simulink model "Simulink_DC_MG_4DGs_4Lines"  (R2024a)
settings: Solver=VariableStepAuto  StartTime=0.0  StopTime=10  RelTol=1e-3
InitFcn:
  | % In your simulation loop or callback function
  | for l = 1:numOfLines
  |     % Generate resistance disturbance (10% variation)
  |     delta_R_l = 0.1 * randn() * Line{l}.R;
  | 
  |     % Update the line resistance with disturbance
  |     Line{l}.R_disturbed = Line{l}.R + delta_R_l;
  | 
  |     % Use this disturbed value in your simulation equations
  |     % L_l * dI_l/dt = -Line{l}.R_disturbed * I_l + (V_i - V_j)
  | end
values from neighbouring files (symbols this model uses):
  Is = value(Is)    [implementTheorem1.m]    (also in implementTheorem1_Obj.m; implementTheorem1_debug.m = []; implementTheorem1_minLoss.m)
  K = sdpvar(1, 3, 'full')    [ComputePassivityForDGs.m]
  l = lines(k, 2)    [generatePhysicalTopology.m]    (also in ploting.m = legend({'\bf With Disturbance'},     'Location','southeast',)
  numOfDGs = size(B_il,1)    [centralizedLocalControlDesign.m]    (also in generateCommunicationTopology.m = size(coords, 1); globalControlDesign.m = size(B_il, 1); verifyControlConditions.m)
undefined symbols (not defined in the file or in its folder): Current_Load_activation, current_variance, D_Activation, DC_Activation, DG, LC_Activation, Line, line_variance, PlugIn, PlugOut, SS_Activation, V_nom, V_ref, voltage_variance
libraries: spsSeriesRLCBranchLib x28, spsControlledCurrentSourceLib x12, spsCurrentMeasurementLib x8, simulink x4, spsIdealSwitchLib x4, spsStairGeneratorLib x4, spsControlledVoltageSourceLib x4, spsDCVoltageSourceLib x4, spsDiodeLib x4, spsIGBTLib x4, spsVoltageMeasurementLib x4, spspowerguiLib x1
(part 1 of 2)
settings Model: Creator=najaf  LastModifiedBy=najaf
settings RTWCC: GPUComputeCapability=3.5

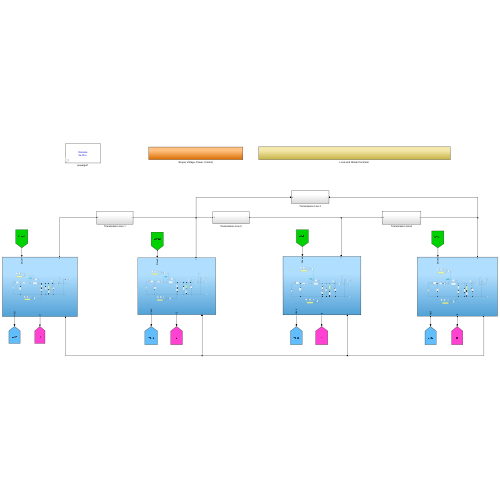
[thumbnail: Simulink's stored preview of the top-level diagram]
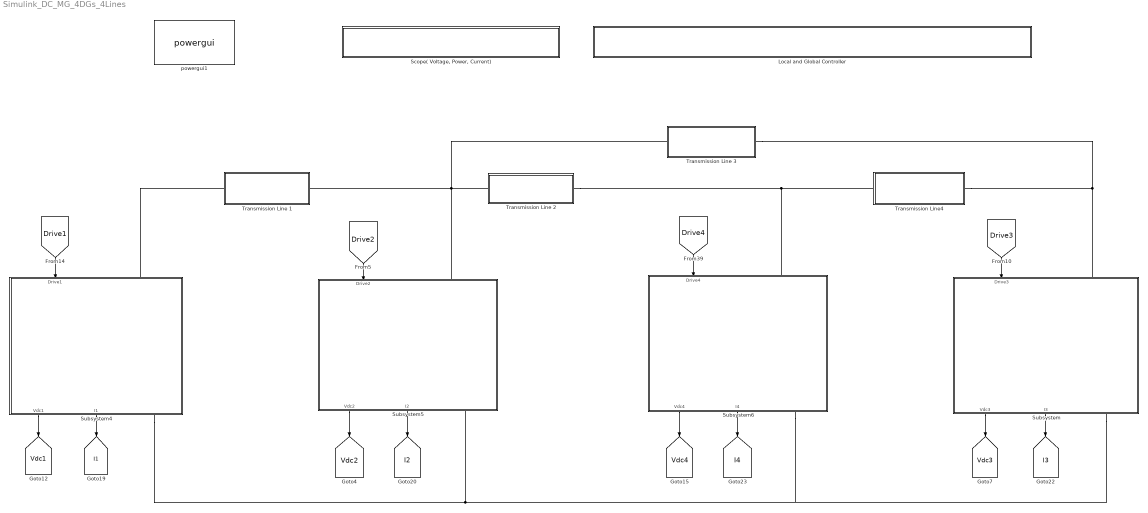
== system Simulink_DC_MG_4DGs_4Lines ==
  "Local and Global Controller " : Subsystem
  "Scope( Voltage, Power, Current)" : Subsystem
  Subsystem : Subsystem
      settings: PortSchema="{\"entries\":[{\"content\":{\"sides\":[{\"content\":{},\"type\":\"ConnectorPlacement.EquallySpacedRectSide\",\"uuid\":\"08b51d35-5d4f-4d5f-a5b0-37344ba45088\"},{\"content\":{\"side\":\"RIGHT\"},\"type\":\"ConnectorPlacement.EquallySpacedRectSide\",\"uuid\":\"3324977a-6e34-487c-ade0-88e1bff4bebb\"},{\"content\":{\"connectorIds\":[\"In1\",\"LConn1\"],\"side\":\"TOP\"},\"type\":\"ConnectorPlacement.EquallySpacedRectSide\",\"uuid\":\"e322db0d-0a35-4471-b922-f546e4cab97b\"},{\"content\":{\"connectorIds\":[\"Out1\",\"Out2\",\"RConn1\"],\"side\":\"BOTTOM\"},\"type\":\"ConnectorPlacement.EquallySpacedRectSide\",\"uuid\":\"57a428a6-4844-4d68-bda7-c5e0dfb814f7\"}]},\"type\":\"ConnectorPlacement.EquallySpacedConnector\",\"uuid\":\"93cb8cb8-3b8c-4430-b1f3-cf7722d9fa22\"}],\"packageUris\":[\"http://schema.mathworks.com/mf0/Connector/R2020b\"],\"version\":\"1.0\"}"
  Subsystem4 : Subsystem
      settings: PortSchema="{\"entries\":[{\"content\":{\"sides\":[{\"content\":{},\"type\":\"ConnectorPlacement.EquallySpacedRectSide\",\"uuid\":\"764b3ce9-8ebc-4171-9263-333df0dfe6fc\"},{\"content\":{\"side\":\"RIGHT\"},\"type\":\"ConnectorPlacement.EquallySpacedRectSide\",\"uuid\":\"c1e9d8a4-dae3-47b0-883a-539aeb69869c\"},{\"content\":{\"connectorIds\":[\"In1\",\"LConn1\"],\"side\":\"TOP\"},\"type\":\"ConnectorPlacement.EquallySpacedRectSide\",\"uuid\":\"bcad0197-72c7-4543-a9ab-ea7942b9cd59\"},{\"content\":{\"connectorIds\":[\"Out1\",\"Out2\",\"RConn1\"],\"side\":\"BOTTOM\"},\"type\":\"ConnectorPlacement.EquallySpacedRectSide\",\"uuid\":\"beb0f75b-103e-4e06-b52f-abd8ae36630a\"}]},\"type\":\"ConnectorPlacement.EquallySpacedConnector\",\"uuid\":\"3998def4-aed0-48b8-bc2a-5ab2d5ec9fd3\"}],\"packageUris\":[\"http://schema.mathworks.com/mf0/Connector/R2020b\"],\"version\":\"1.0\"}"
  Subsystem5 : Subsystem
      settings: PortSchema="{\"entries\":[{\"content\":{\"sides\":[{\"content\":{},\"type\":\"ConnectorPlacement.EquallySpacedRectSide\",\"uuid\":\"08b51d35-5d4f-4d5f-a5b0-37344ba45088\"},{\"content\":{\"side\":\"RIGHT\"},\"type\":\"ConnectorPlacement.EquallySpacedRectSide\",\"uuid\":\"3324977a-6e34-487c-ade0-88e1bff4bebb\"},{\"content\":{\"connectorIds\":[\"In1\",\"LConn1\"],\"side\":\"TOP\"},\"type\":\"ConnectorPlacement.EquallySpacedRectSide\",\"uuid\":\"e322db0d-0a35-4471-b922-f546e4cab97b\"},{\"content\":{\"connectorIds\":[\"Out1\",\"Out2\",\"RConn1\"],\"side\":\"BOTTOM\"},\"type\":\"ConnectorPlacement.EquallySpacedRectSide\",\"uuid\":\"f52eba1b-ac2a-4c74-a10c-8b92ab05ae45\"}]},\"type\":\"ConnectorPlacement.EquallySpacedConnector\",\"uuid\":\"93cb8cb8-3b8c-4430-b1f3-cf7722d9fa22\"}],\"packageUris\":[\"http://schema.mathworks.com/mf0/Connector/R2020b\"],\"version\":\"1.0\"}"
  Subsystem6 : Subsystem
      settings: PortSchema="{\"entries\":[{\"content\":{\"sides\":[{\"content\":{},\"type\":\"ConnectorPlacement.EquallySpacedRectSide\",\"uuid\":\"764b3ce9-8ebc-4171-9263-333df0dfe6fc\"},{\"content\":{\"side\":\"RIGHT\"},\"type\":\"ConnectorPlacement.EquallySpacedRectSide\",\"uuid\":\"c1e9d8a4-dae3-47b0-883a-539aeb69869c\"},{\"content\":{\"connectorIds\":[\"In1\",\"LConn1\"],\"side\":\"TOP\"},\"type\":\"ConnectorPlacement.EquallySpacedRectSide\",\"uuid\":\"bcad0197-72c7-4543-a9ab-ea7942b9cd59\"},{\"content\":{\"connectorIds\":[\"Out1\",\"Out2\",\"RConn1\"],\"side\":\"BOTTOM\"},\"type\":\"ConnectorPlacement.EquallySpacedRectSide\",\"uuid\":\"43195860-d6e2-4bd9-a504-1cc2264ea7f4\"}]},\"type\":\"ConnectorPlacement.EquallySpacedConnector\",\"uuid\":\"3998def4-aed0-48b8-bc2a-5ab2d5ec9fd3\"}],\"packageUris\":[\"http://schema.mathworks.com/mf0/Connector/R2020b\"],\"version\":\"1.0\"}"
  Transmission Line 1 : Subsystem
  Transmission Line 2 : Subsystem
  Transmission Line 3 : Subsystem
  Transmission Line4 : Subsystem
  powergui1 : spspowerguiLib/powergui  Priority=1  SimulationMode=Discrete  SampleTime=5e-5  frequency=60  Iterations=50  frequencyindice=0  Pbase=100e6  ErrMax=1e-4  UnitsV=kV  UnitsW=MW  buscounter=0  FunctionMessages=off  echomessages=off  EnableUseOfTLC=off  CurrentSourceSwitches=off  DisableSnubberDevices=off  DisableRonSwitches=off  DisableVfSwitches=off  DisplayEquations=off  AutomaticDiscreteSolvers=off  SolverType=Tustin/Backward Euler (TBE)  Interpol=off  ExternalGateDelay=off  methode=off  Ts=100  x0status=blocks  SPID=on  SwTol=0  HookPort=off  NonlinearTolerance=1e-4  nMaxIteration=100  ContinueOnMaxIteration=off  RestoreLinks=warning  ResistiveCurrentMeasurement=off  Frange=[0:2:500]  Ylog=off  Xlog=on  ShowGrid=off  save=off  variable=ZData  structure=0  ZoomFFT=off  StartTime=0.0  cycles=1  DisplayStyle=1  fundamental=60  FreqAxis=off  MaxFrequency=1000  frequencyindicesteady=1  RmsSteady=1  display=off
  tag scope: I1=global, I2=global, I3=global, I4=global, Vdc1=global, Vdc2=global, Vdc3=global, Vdc4=global
  wires:
  [Drive4] -> Subsystem6/1(Drive4)
  Subsystem6/1(Vdc4) -> [Vdc4]
  Subsystem6/2(I4) -> [I4]
  [Drive1] -> Subsystem4/1(Drive1)
  Subsystem4/1(Vdc1) -> [Vdc1]
  Subsystem4/2(I1) -> [I1]
  [Drive2] -> Subsystem5/1(Drive2)
  [Drive3] -> Subsystem/1(Drive3)
  Subsystem/2(I3) -> [I3]
  Subsystem/1(Vdc3) -> [Vdc3]
  Subsystem5/1(Vdc2) -> [Vdc2]
  Subsystem5/2(I2) -> [I2]
  connections:
  Transmission Line 1/LConn1 -- Subsystem4/LConn1
  Transmission Line4/RConn1 -- Subsystem/LConn1 -- Transmission Line 3/RConn1
  Subsystem4/RConn1 -- Subsystem5/RConn1 -- Subsystem6/RConn1 -- Subsystem/RConn1
  Transmission Line 2/RConn1 -- Subsystem6/LConn1 -- Transmission Line4/LConn1
  Transmission Line 2/LConn1 -- Transmission Line 3/LConn1 -- Subsystem5/LConn1 -- Transmission Line 1/RConn1

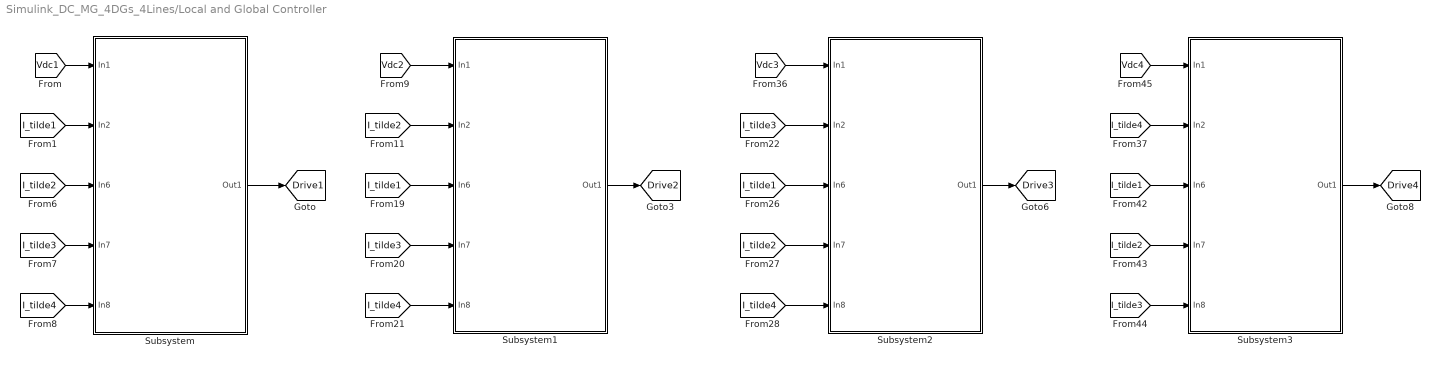
== system Simulink_DC_MG_4DGs_4Lines/Local and Global Controller  ==
  Subsystem : Subsystem
  Subsystem1 : Subsystem
  Subsystem2 : Subsystem
  Subsystem3 : Subsystem
  tag scope: Drive1=global, Drive2=global, Drive3=global, Drive4=global
  wires:
  [I_tilde3] -> Subsystem3/5(In8)
  Subsystem3/1(Out1) -> [Drive4]
  [I_tilde1] -> Subsystem3/3(In6)
  [I_tilde2] -> Subsystem3/4(In7)
  [I_tilde4] -> Subsystem1/5(In8)
  [I_tilde4] -> Subsystem3/2(In2)
  [Vdc4] -> Subsystem3/1(In1)
  [I_tilde1] -> Subsystem1/3(In6)
  [Vdc2] -> Subsystem1/1(In1)
  [I_tilde3] -> Subsystem1/4(In7)
  Subsystem1/1(Out1) -> [Drive2]
  [I_tilde2] -> Subsystem1/2(In2)
  Subsystem2/1(Out1) -> [Drive3]
  [I_tilde3] -> Subsystem2/2(In2)
  [I_tilde4] -> Subsystem2/5(In8)
  [I_tilde1] -> Subsystem2/3(In6)
  [Vdc3] -> Subsystem2/1(In1)
  [I_tilde2] -> Subsystem2/4(In7)
  Subsystem/1(Out1) -> [Drive1]
  [I_tilde2] -> Subsystem/3(In6)
  [I_tilde3] -> Subsystem/4(In7)
  [I_tilde4] -> Subsystem/5(In8)
  [Vdc1] -> Subsystem/1(In1)
  [I_tilde1] -> Subsystem/2(In2)

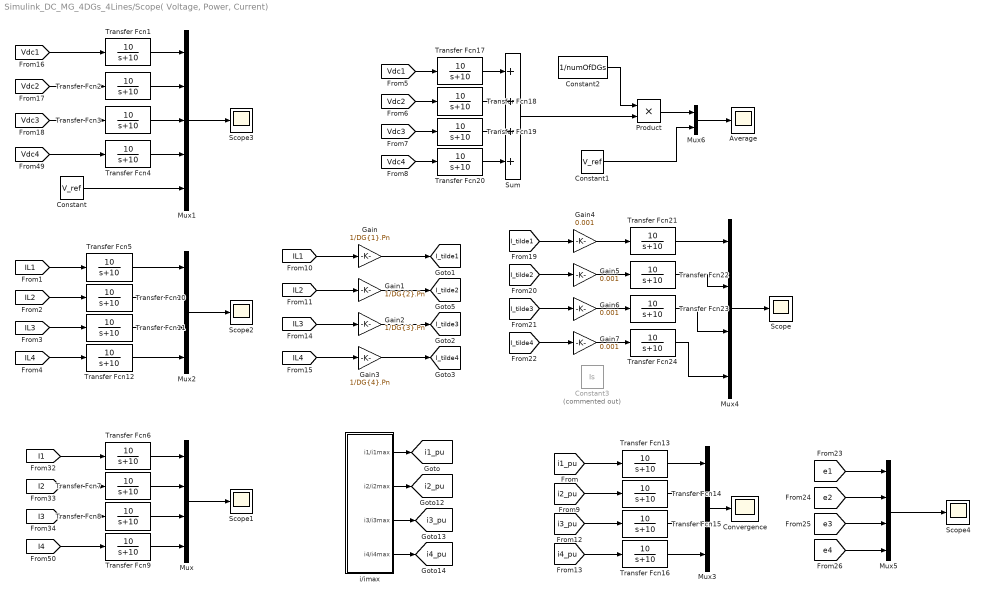
== system Simulink_DC_MG_4DGs_4Lines/Scope( Voltage, Power, Current) ==
  Average : Scope
  Constant : Constant  Value=V_ref
  Constant1 : Constant  Value=V_ref
  Constant2 : Constant  Value=1/numOfDGs
  Constant3 : Constant  Commented=on  Value=Is
  Convergence : Scope
  Gain : Gain  Gain=1/DG{1}.Pn
  Gain1 : Gain  Gain=1/DG{2}.Pn
  Gain2 : Gain  Gain=1/DG{3}.Pn
  Gain3 : Gain  Gain=1/DG{4}.Pn
  Gain{4..7} (4 alike) : Gain  Gain=0.001
  Mux{,2..5} (5 alike) : Mux
  Mux1 : Mux  Inputs=5
  Mux6 : Mux  Inputs=2
  Product : Product
  Scope{,1..4} (5 alike) : Scope
  Sum : Sum  Inputs=++++
  Transfer Fcn{1..24} (24 alike) : TransferFcn  Numerator=[10]  Denominator=[1 10]
  i/imax : Subsystem
  tag scope: I_tilde1=global, I_tilde2=global, I_tilde3=global, I_tilde4=global, i1_pu=global, i2_pu=global, i3_pu=global, i4_pu=global
  wires:
  Mux/1 -> Scope1/1
  Mux1/1 -> Scope3/1
  [Vdc1] -> Transfer Fcn1/1
  [Vdc2] -> Transfer Fcn2/1
  [Vdc3] -> Transfer Fcn3/1
  [Vdc4] -> Transfer Fcn4/1
  [I1] -> Transfer Fcn6/1
  [I2] -> Transfer Fcn7/1
  [I3] -> Transfer Fcn8/1
  [I4] -> Transfer Fcn9/1
  Constant/1 -> Mux1/5
  [IL4] -> Transfer Fcn12/1
  [IL3] -> Transfer Fcn11/1
  [IL2] -> Transfer Fcn10/1
  [IL1] -> Transfer Fcn5/1
  Mux2/1 -> Scope2/1
  Transfer Fcn6/1 -> Mux/1
  Transfer Fcn7/1 -> Mux/2
  Transfer Fcn8/1 -> Mux/3
  Transfer Fcn9/1 -> Mux/4
  i/imax/1(i1/i1max) -> [i1_pu]
  i/imax/3(i3/i3max) -> [i3_pu]
  i/imax/4(i4/i4max) -> [i4_pu]
  i/imax/2(i2/i2max) -> [i2_pu]
  [i2_pu] -> Transfer Fcn14/1
  [i3_pu] -> Transfer Fcn15/1
  Mux3/1 -> Convergence/1
  [i4_pu] -> Transfer Fcn16/1
  [i1_pu] -> Transfer Fcn13/1
  Transfer Fcn13/1 -> Mux3/1
  Transfer Fcn14/1 -> Mux3/2
  Transfer Fcn15/1 -> Mux3/3
  Transfer Fcn16/1 -> Mux3/4
  [Vdc4] -> Transfer Fcn20/1
  [Vdc3] -> Transfer Fcn19/1
  Transfer Fcn18/1 -> Sum/2
  Transfer Fcn19/1 -> Sum/3
  [Vdc2] -> Transfer Fcn18/1
  Transfer Fcn20/1 -> Sum/4
  Constant2/1 -> Product/1
  [Vdc1] -> Transfer Fcn17/1
  Sum/1 -> Product/2
  Transfer Fcn17/1 -> Sum/1
  Transfer Fcn1/1 -> Mux1/1
  Transfer Fcn2/1 -> Mux1/2
  Transfer Fcn3/1 -> Mux1/3
  Transfer Fcn4/1 -> Mux1/4
  Gain/1 -> [I_tilde1]
  [IL1] -> Gain/1
  Gain1/1 -> [I_tilde2]
  [IL2] -> Gain1/1
  [IL3] -> Gain2/1
  Gain2/1 -> [I_tilde3]
  Gain3/1 -> [I_tilde4]
  [IL4] -> Gain3/1
  [I_tilde1] -> Gain4/1
  [I_tilde2] -> Gain5/1
  [I_tilde3] -> Gain6/1
  [I_tilde4] -> Gain7/1
  Gain4/1 -> Transfer Fcn21/1
  Gain5/1 -> Transfer Fcn22/1
  Gain6/1 -> Transfer Fcn23/1
  Gain7/1 -> Transfer Fcn24/1
  Transfer Fcn5/1 -> Mux2/1
  Transfer Fcn10/1 -> Mux2/2
  Transfer Fcn11/1 -> Mux2/3
  Transfer Fcn12/1 -> Mux2/4
  [e1] -> Mux5/1
  [e2] -> Mux5/2
  [e3] -> Mux5/3
  [e4] -> Mux5/4
  Mux5/1 -> Scope4/1
  Transfer Fcn24/1 -> Mux4/4
  Transfer Fcn23/1 -> Mux4/3
  Transfer Fcn22/1 -> Mux4/2
  Transfer Fcn21/1 -> Mux4/1
  Mux4/1 -> Scope/1
  Product/1 -> Mux6/1
  Constant1/1 -> Mux6/2
  Mux6/1 -> Average/1

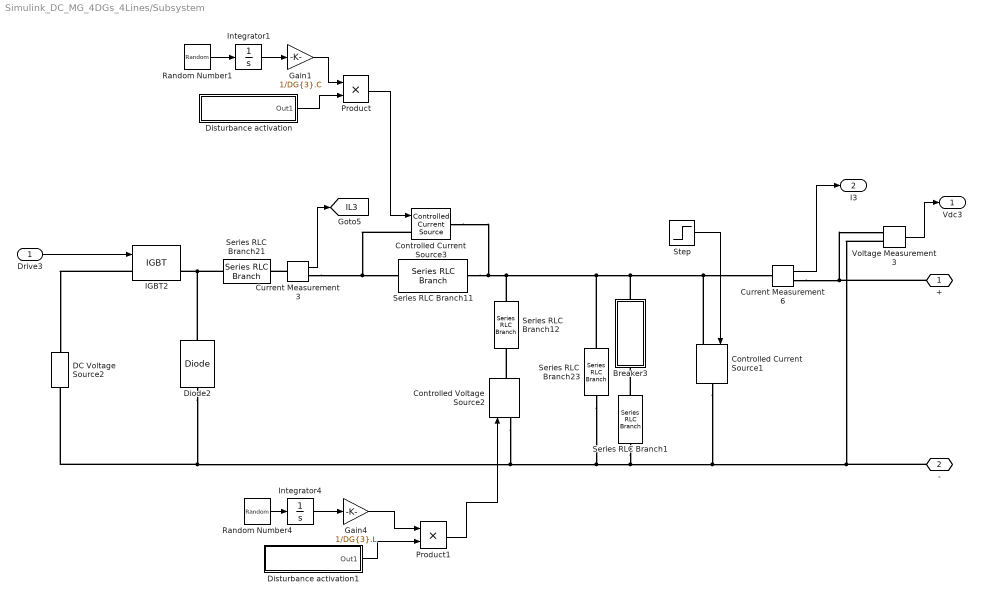
== system Simulink_DC_MG_4DGs_4Lines/Subsystem ==
  Drive3 : Inport
  Breaker3 : Subsystem
  Controlled Current Source1 : spsControlledCurrentSourceLib/Controlled Current Source  Initialize=on  Source_Type=DC  Amplitude=DG{2}.IL  Phase=0  Frequency=0  Measurements=None
  Controlled Current Source3 : spsControlledCurrentSourceLib/Controlled Current Source  Initialize=on  Source_Type=DC  Amplitude=0  Phase=0  Frequency=0  Measurements=None
  Controlled Voltage Source2 : spsControlledVoltageSourceLib/Controlled Voltage Source  Initialize=on  Source_Type=DC  Amplitude=0  Phase=0  Frequency=0  Measurements=None
  Current Measurement3 : spsCurrentMeasurementLib/Current Measurement  PhasorSimulation=off  OutputType=Complex  PSBequivalent=0
  Current Measurement6 : spsCurrentMeasurementLib/Current Measurement  PhasorSimulation=off  OutputType=Complex  PSBequivalent=0
  DC Voltage Source2 : spsDCVoltageSourceLib/DC Voltage Source  Amplitude=V_nom  Measurements=None
  Diode2 : spsDiodeLib/Diode  Ron=0.001  Lon=0  Vf=0.8  IC=0  UseSnubber=off  Rs=500  Cs=0  Measurements=off
  Disturbance activation : Subsystem
  Disturbance activation1 : Subsystem
  Gain1 : Gain  Gain=1/DG{3}.C
  Gain4 : Gain  Gain=1/DG{3}.L
  IGBT2 : spsIGBTLib/IGBT  Ron=0.001  Lon=0  Vf=1  Tf=1e-6  Tt=2e-6  IC=0  Rs=1e5  Cs=inf  Measurements=on
  Integrator1 : Integrator
  Integrator4 : Integrator
  Product : Product
  Product1 : Product
  Random Number1 : RandomNumber  Variance=current_variance  SampleTime=0.0001
  Random Number4 : RandomNumber  Variance=voltage_variance  SampleTime=0.0001
  Series RLC Branch1 : spsSeriesRLCBranchLib/Series RLC Branch  LConnTagsString=__new0  RConnTagsString=__new0  BranchType=R  Resistance=DG{3}.Y  Inductance=1e-2  SetiL0=off  InitialCurrent=0  Capacitance=2.2e-3  Setx0=off  InitialVoltage=0  Measurements=None
  Series RLC Branch11 : spsSeriesRLCBranchLib/Series RLC Branch  LConnTagsString=__new0  RConnTagsString=__new0  BranchType=L  Resistance=1  Inductance=DG{3}.L  SetiL0=off  InitialCurrent=0  Capacitance=1e-6  Setx0=off  InitialVoltage=0  Measurements=Branch current
  Series RLC Branch12 : spsSeriesRLCBranchLib/Series RLC Branch  LConnTagsString=__new0  RConnTagsString=__new0  BranchType=C  Resistance=1  Inductance=1e-2  SetiL0=off  InitialCurrent=0  Capacitance=DG{4}.C  Setx0=off  InitialVoltage=0  Measurements=None
  Series RLC Branch21 : spsSeriesRLCBranchLib/Series RLC Branch  LConnTagsString=__new0  RConnTagsString=__new0  BranchType=R  Resistance=DG{3}.R  Inductance=1e-2  SetiL0=off  InitialCurrent=0  Capacitance=2.2e-3  Setx0=off  InitialVoltage=0  Measurements=None
  Series RLC Branch23 : spsSeriesRLCBranchLib/Series RLC Branch  LConnTagsString=__new0  RConnTagsString=__new0  BranchType=R  Resistance=DG{3}.Y  Inductance=1e-2  SetiL0=off  InitialCurrent=0  Capacitance=2.2e-3  Setx0=off  InitialVoltage=0  Measurements=None
  Step : Step  Time=Current_Load_activation  SampleTime=0
  Voltage Measurement3 : spsVoltageMeasurementLib/Voltage Measurement  PhasorSimulation=off  OutputType=Complex  PSBequivalent=0
  + : PMIOPort  Side=Left
  - : PMIOPort  Port=2  Side=Right
  Vdc3 : Outport
  I3 : Outport  Port=2
  tag scope: IL3=global
  wires:
  Current Measurement3/1 -> [IL3]
  Drive3/1 -> IGBT2/1
  Current Measurement6/1 -> I3/1
  Voltage Measurement3/1 -> Vdc3/1
  Integrator1/1 -> Gain1/1
  Random Number4/1 -> Integrator4/1
  Integrator4/1 -> Gain4/1
  Random Number1/1 -> Integrator1/1
  Gain1/1 -> Product/1
  Disturbance activation/1(Out1) -> Product/2
  Product/1 -> Controlled Current Source3/1
  Gain4/1 -> Product1/1
  Disturbance activation1/1(Out1) -> Product1/2
  Product1/1 -> Controlled Voltage Source2/1
  Step/1 -> Controlled Current Source1/1
  connections:
  Series RLC Branch12/LConn1 -- Controlled Current Source3/RConn1 -- Series RLC Branch11/RConn1 -- Series RLC Branch23/LConn1 -- Controlled Current Source1/LConn1 -- Current Measurement6/LConn1 -- Breaker3/RConn1
  Voltage Measurement3/LConn2 -- Controlled Current Source1/RConn1 -- Controlled Voltage Source2/LConn1 -- Diode2/LConn1 -- DC Voltage Source2/LConn1 -- Series RLC Branch23/RConn1 -- Series RLC Branch1/RConn1 -- -/RConn1
  Current Measurement6/RConn1 -- +/RConn1 -- Voltage Measurement3/LConn1
  Diode2/RConn1 -- Series RLC Branch21/RConn1 -- IGBT2/RConn1
  IGBT2/LConn1 -- DC Voltage Source2/RConn1
  Series RLC Branch1/LConn1 -- Breaker3/LConn1
  Current Measurement3/RConn1 -- Controlled Current Source3/LConn1 -- Series RLC Branch11/LConn1
  Current Measurement3/LConn1 -- Series RLC Branch21/LConn1
  Controlled Voltage Source2/RConn1 -- Series RLC Branch12/RConn1

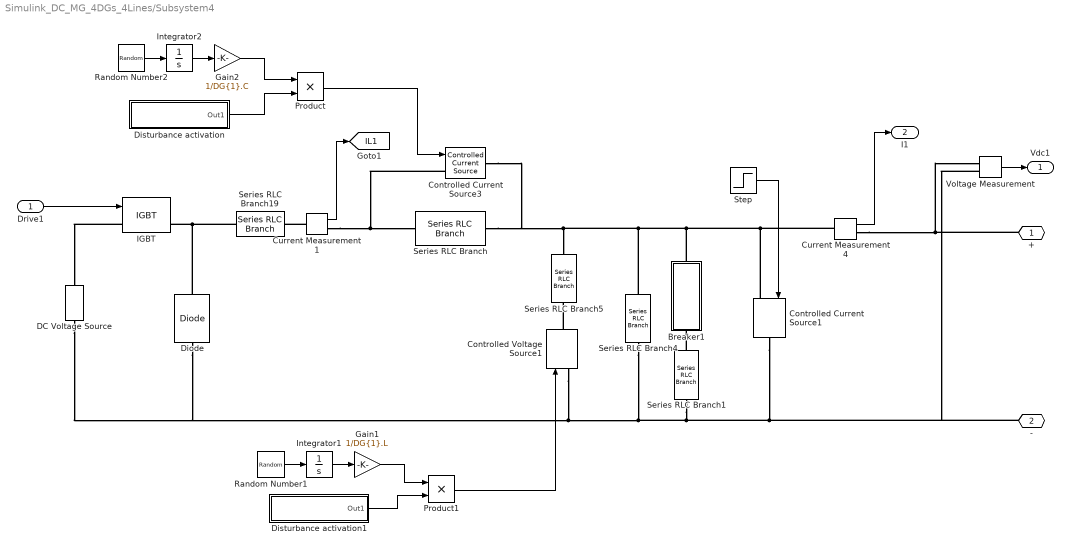
== system Simulink_DC_MG_4DGs_4Lines/Subsystem4 ==
  Drive1 : Inport
  Breaker1 : Subsystem
  Controlled Current Source1 : spsControlledCurrentSourceLib/Controlled Current Source  Initialize=on  Source_Type=DC  Amplitude=DG{1}.IL  Phase=0  Frequency=0  Measurements=None
  Controlled Current Source3 : spsControlledCurrentSourceLib/Controlled Current Source  Initialize=on  Source_Type=DC  Amplitude=0  Phase=0  Frequency=0  Measurements=None
  Controlled Voltage Source1 : spsControlledVoltageSourceLib/Controlled Voltage Source  Initialize=on  Source_Type=DC  Amplitude=0  Phase=0  Frequency=0  Measurements=None
  Current Measurement1 : spsCurrentMeasurementLib/Current Measurement  PhasorSimulation=off  OutputType=Complex  PSBequivalent=0
  Current Measurement4 : spsCurrentMeasurementLib/Current Measurement  PhasorSimulation=off  OutputType=Complex  PSBequivalent=0
  DC Voltage Source : spsDCVoltageSourceLib/DC Voltage Source  Amplitude=V_nom  Measurements=None
  Diode : spsDiodeLib/Diode  Ron=0.001  Lon=0  Vf=0.8  IC=0  UseSnubber=off  Rs=500  Cs=0  Measurements=off
  Disturbance activation : Subsystem
  Disturbance activation1 : Subsystem
  Gain1 : Gain  Gain=1/DG{1}.L
  Gain2 : Gain  Gain=1/DG{1}.C
  IGBT : spsIGBTLib/IGBT  Ron=0.001  Lon=0  Vf=1  Tf=1e-6  Tt=2e-6  IC=0  Rs=1e5  Cs=inf  Measurements=on
  Integrator1 : Integrator
  Integrator2 : Integrator
  Product : Product
  Product1 : Product
  Random Number1 : RandomNumber  Variance=voltage_variance  SampleTime=0.0001
  Random Number2 : RandomNumber  Variance=current_variance  SampleTime=0.0001
  Series RLC Branch : spsSeriesRLCBranchLib/Series RLC Branch  LConnTagsString=__new0  RConnTagsString=__new0  BranchType=L  Resistance=1  Inductance=DG{1}.L  SetiL0=off  InitialCurrent=0  Capacitance=1e-6  Setx0=off  InitialVoltage=0  Measurements=Branch current
  Series RLC Branch1 : spsSeriesRLCBranchLib/Series RLC Branch  LConnTagsString=__new0  RConnTagsString=__new0  BranchType=R  Resistance=DG{1}.Y  Inductance=1e-2  SetiL0=off  InitialCurrent=0  Capacitance=2.2e-3  Setx0=off  InitialVoltage=0  Measurements=None
  Series RLC Branch19 : spsSeriesRLCBranchLib/Series RLC Branch  LConnTagsString=__new0  RConnTagsString=__new0  BranchType=R  Resistance=DG{1}.R  Inductance=1e-2  SetiL0=off  InitialCurrent=0  Capacitance=2.2e-3  Setx0=off  InitialVoltage=0  Measurements=None
  Series RLC Branch4 : spsSeriesRLCBranchLib/Series RLC Branch  LConnTagsString=__new0  RConnTagsString=__new0  BranchType=R  Resistance=DG{1}.Y  Inductance=1e-2  SetiL0=off  InitialCurrent=0  Capacitance=2.2e-3  Setx0=off  InitialVoltage=0  Measurements=None
  Series RLC Branch5 : spsSeriesRLCBranchLib/Series RLC Branch  LConnTagsString=__new0  RConnTagsString=__new0  BranchType=C  Resistance=1  Inductance=1e-2  SetiL0=off  InitialCurrent=0  Capacitance=DG{1}.C  Setx0=off  InitialVoltage=0  Measurements=None
  Step : Step  Time=Current_Load_activation  SampleTime=0
  Voltage Measurement : spsVoltageMeasurementLib/Voltage Measurement  PhasorSimulation=off  OutputType=Complex  PSBequivalent=0
  + : PMIOPort  Side=Left
  - : PMIOPort  Port=2  Side=Right
  Vdc1 : Outport
  I1 : Outport  Port=2
  tag scope: IL1=global
  wires:
  Current Measurement1/1 -> [IL1]
  Current Measurement4/1 -> I1/1
  Voltage Measurement/1 -> Vdc1/1
  Drive1/1 -> IGBT/1
  Integrator2/1 -> Gain2/1
  Random Number2/1 -> Integrator2/1
  Integrator1/1 -> Gain1/1
  Random Number1/1 -> Integrator1/1
  Gain2/1 -> Product/1
  Disturbance activation/1(Out1) -> Product/2
  Product/1 -> Controlled Current Source3/1
  Gain1/1 -> Product1/1
  Disturbance activation1/1(Out1) -> Product1/2
  Product1/1 -> Controlled Voltage Source1/1
  Step/1 -> Controlled Current Source1/1
  connections:
  Current Measurement4/RConn1 -- +/RConn1 -- Voltage Measurement/LConn1
  -/RConn1 -- Voltage Measurement/LConn2 -- Controlled Current Source1/RConn1 -- Series RLC Branch1/RConn1 -- Controlled Voltage Source1/LConn1 -- Diode/LConn1 -- DC Voltage Source/LConn1 -- Series RLC Branch4/RConn1
  Current Measurement4/LConn1 -- Controlled Current Source1/LConn1 -- Breaker1/RConn1 -- Series RLC Branch4/LConn1 -- Controlled Current Source3/RConn1 -- Series RLC Branch/RConn1 -- Series RLC Branch5/LConn1
  IGBT/LConn1 -- DC Voltage Source/RConn1
  Diode/RConn1 -- Series RLC Branch19/RConn1 -- IGBT/RConn1
  Series RLC Branch1/LConn1 -- Breaker1/LConn1
  Current Measurement1/RConn1 -- Controlled Current Source3/LConn1 -- Series RLC Branch/LConn1
  Current Measurement1/LConn1 -- Series RLC Branch19/LConn1
  Controlled Voltage Source1/RConn1 -- Series RLC Branch5/RConn1

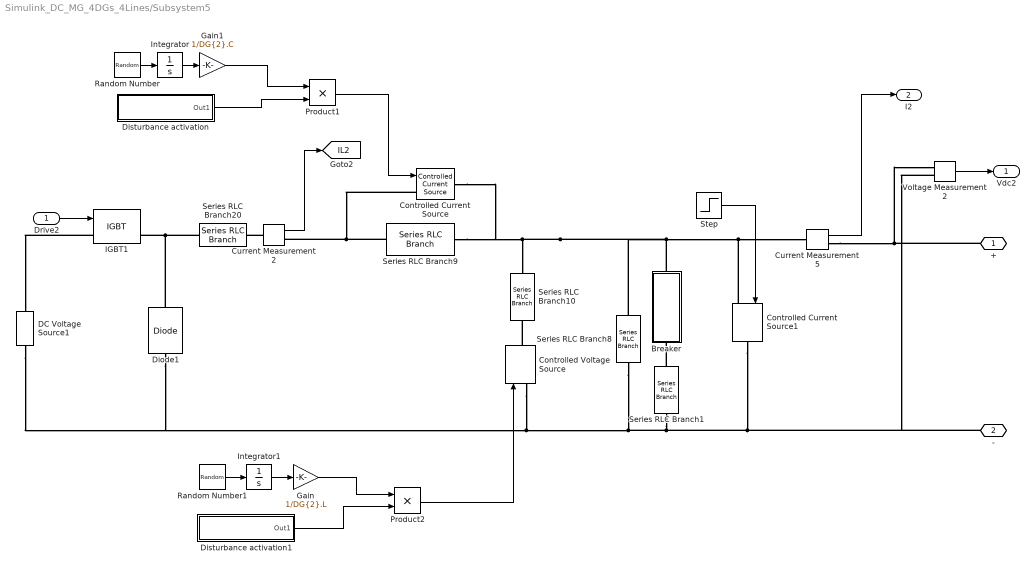
== system Simulink_DC_MG_4DGs_4Lines/Subsystem5 ==
  Drive2 : Inport
  Breaker : Subsystem
  Controlled Current Source : spsControlledCurrentSourceLib/Controlled Current Source  Initialize=on  Source_Type=DC  Amplitude=0  Phase=0  Frequency=0  Measurements=None
  Controlled Current Source1 : spsControlledCurrentSourceLib/Controlled Current Source  Initialize=on  Source_Type=DC  Amplitude=DG{4}.IL  Phase=0  Frequency=0  Measurements=None
  Controlled Voltage Source : spsControlledVoltageSourceLib/Controlled Voltage Source  Initialize=on  Source_Type=DC  Amplitude=0  Phase=0  Frequency=0  Measurements=None
  Current Measurement2 : spsCurrentMeasurementLib/Current Measurement  PhasorSimulation=off  OutputType=Complex  PSBequivalent=0
  Current Measurement5 : spsCurrentMeasurementLib/Current Measurement  PhasorSimulation=off  OutputType=Complex  PSBequivalent=0
  DC Voltage Source1 : spsDCVoltageSourceLib/DC Voltage Source  Amplitude=V_nom  Measurements=None
  Diode1 : spsDiodeLib/Diode  Ron=0.001  Lon=0  Vf=0.8  IC=0  UseSnubber=off  Rs=500  Cs=0  Measurements=off
  Disturbance activation : Subsystem
  Disturbance activation1 : Subsystem
  Gain : Gain  Gain=1/DG{2}.L
  Gain1 : Gain  Gain=1/DG{2}.C
  IGBT1 : spsIGBTLib/IGBT  Ron=0.001  Lon=0  Vf=1  Tf=1e-6  Tt=2e-6  IC=0  Rs=1e5  Cs=inf  Measurements=on
  Integrator : Integrator
  Integrator1 : Integrator
  Product1 : Product
  Product2 : Product
  Random Number : RandomNumber  Variance=current_variance  SampleTime=0.0001
  Random Number1 : RandomNumber  Variance=voltage_variance  SampleTime=0.0001
  Series RLC Branch1 : spsSeriesRLCBranchLib/Series RLC Branch  LConnTagsString=__new0  RConnTagsString=__new0  BranchType=R  Resistance=DG{2}.Y  Inductance=1e-2  SetiL0=off  InitialCurrent=0  Capacitance=2.2e-3  Setx0=off  InitialVoltage=0  Measurements=None
  Series RLC Branch10 : spsSeriesRLCBranchLib/Series RLC Branch  LConnTagsString=__new0  RConnTagsString=__new0  BranchType=C  Resistance=1  Inductance=1e-2  SetiL0=off  InitialCurrent=0  Capacitance=DG{2}.C  Setx0=off  InitialVoltage=0  Measurements=None
  Series RLC Branch20 : spsSeriesRLCBranchLib/Series RLC Branch  LConnTagsString=__new0  RConnTagsString=__new0  BranchType=R  Resistance=DG{2}.R  Inductance=1e-2  SetiL0=off  InitialCurrent=0  Capacitance=2.2e-3  Setx0=off  InitialVoltage=0  Measurements=None
  Series RLC Branch8 : spsSeriesRLCBranchLib/Series RLC Branch  LConnTagsString=__new0  RConnTagsString=__new0  BranchType=R  Resistance=DG{2}.Y  Inductance=1e-2  SetiL0=off  InitialCurrent=0  Capacitance=2.2e-3  Setx0=off  InitialVoltage=0  Measurements=None
  Series RLC Branch9 : spsSeriesRLCBranchLib/Series RLC Branch  LConnTagsString=__new0  RConnTagsString=__new0  BranchType=L  Resistance=1  Inductance=DG{2}.L  SetiL0=off  InitialCurrent=0  Capacitance=1e-6  Setx0=off  InitialVoltage=0  Measurements=Branch current
  Step : Step  Time=Current_Load_activation  SampleTime=0
  Voltage Measurement2 : spsVoltageMeasurementLib/Voltage Measurement  PhasorSimulation=off  OutputType=Complex  PSBequivalent=0
  + : PMIOPort  Side=Left
  - : PMIOPort  Port=2  Side=Right
  Vdc2 : Outport
  I2 : Outport  Port=2
  tag scope: IL2=global
  wires:
  Current Measurement2/1 -> [IL2]
  Drive2/1 -> IGBT1/1
  Current Measurement5/1 -> I2/1
  Voltage Measurement2/1 -> Vdc2/1
  Random Number1/1 -> Integrator1/1
  Random Number/1 -> Integrator/1
  Integrator/1 -> Gain1/1
  Integrator1/1 -> Gain/1
  Disturbance activation/1(Out1) -> Product1/2
  Gain1/1 -> Product1/1
  Product1/1 -> Controlled Current Source/1
  Disturbance activation1/1(Out1) -> Product2/2
  Gain/1 -> Product2/1
  Product2/1 -> Controlled Voltage Source/1
  Step/1 -> Controlled Current Source1/1
  connections:
  Current Measurement5/RConn1 -- Voltage Measurement2/LConn1 -- +/RConn1
  Diode1/RConn1 -- Series RLC Branch20/RConn1 -- IGBT1/RConn1
  Series RLC Branch1/RConn1 -- Controlled Current Source1/RConn1 -- -/RConn1 -- Voltage Measurement2/LConn2 -- Controlled Voltage Source/LConn1 -- DC Voltage Source1/LConn1 -- Diode1/LConn1 -- Series RLC Branch8/RConn1
  IGBT1/LConn1 -- DC Voltage Source1/RConn1
  Series RLC Branch1/LConn1 -- Breaker/LConn1
  Current Measurement2/LConn1 -- Series RLC Branch20/LConn1
  Series RLC Branch9/LConn1 -- Controlled Current Source/LConn1 -- Current Measurement2/RConn1
  Breaker/RConn1 -- Series RLC Branch8/LConn1 -- Controlled Current Source/RConn1 -- Series RLC Branch9/RConn1 -- Series RLC Branch10/LConn1 -- Controlled Current Source1/LConn1 -- Current Measurement5/LConn1
  Controlled Voltage Source/RConn1 -- Series RLC Branch10/RConn1

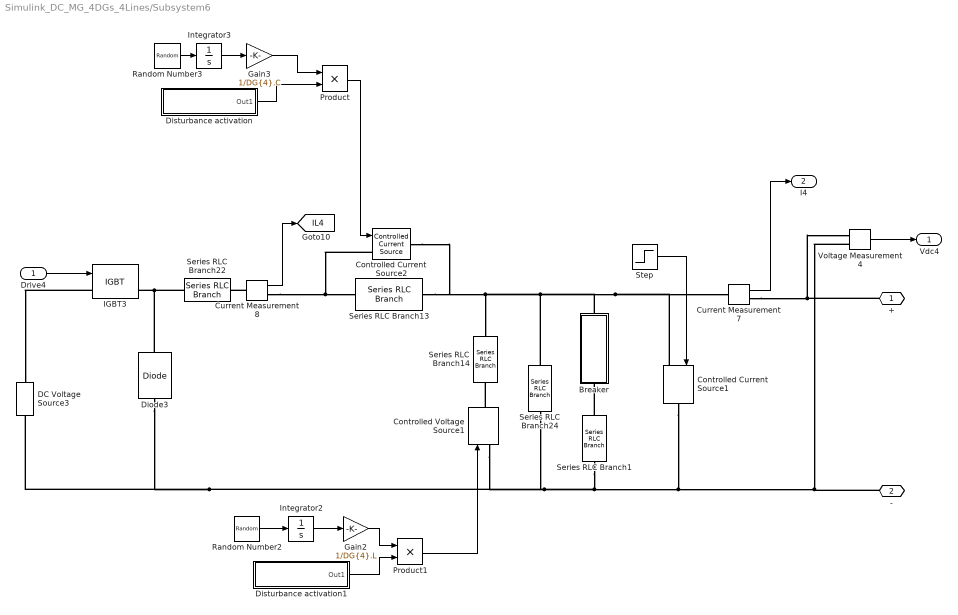
== system Simulink_DC_MG_4DGs_4Lines/Subsystem6 ==
  Drive4 : Inport
  Breaker : Subsystem
  Controlled Current Source1 : spsControlledCurrentSourceLib/Controlled Current Source  Initialize=on  Source_Type=DC  Amplitude=DG{3}.IL  Phase=0  Frequency=0  Measurements=None
  Controlled Current Source2 : spsControlledCurrentSourceLib/Controlled Current Source  Initialize=on  Source_Type=DC  Amplitude=0  Phase=0  Frequency=0  Measurements=None
  Controlled Voltage Source1 : spsControlledVoltageSourceLib/Controlled Voltage Source  Initialize=on  Source_Type=DC  Amplitude=0  Phase=0  Frequency=0  Measurements=None
  Current Measurement7 : spsCurrentMeasurementLib/Current Measurement  PhasorSimulation=off  OutputType=Complex  PSBequivalent=0
  Current Measurement8 : spsCurrentMeasurementLib/Current Measurement  PhasorSimulation=off  OutputType=Complex  PSBequivalent=0
  DC Voltage Source3 : spsDCVoltageSourceLib/DC Voltage Source  Amplitude=V_nom  Measurements=None
  Diode3 : spsDiodeLib/Diode  Ron=0.001  Lon=0  Vf=0.8  IC=0  UseSnubber=off  Rs=500  Cs=0  Measurements=off
  Disturbance activation : Subsystem
  Disturbance activation1 : Subsystem
  Gain2 : Gain  Gain=1/DG{4}.L
  Gain3 : Gain  Gain=1/DG{4}.C
  IGBT3 : spsIGBTLib/IGBT  Ron=0.001  Lon=0  Vf=1  Tf=1e-6  Tt=2e-6  IC=0  Rs=1e5  Cs=inf  Measurements=on
  Integrator2 : Integrator
  Integrator3 : Integrator
  Product : Product
  Product1 : Product
  Random Number2 : RandomNumber  Variance=voltage_variance  SampleTime=0.0001
  Random Number3 : RandomNumber  Variance=current_variance  SampleTime=0.0001
  Series RLC Branch1 : spsSeriesRLCBranchLib/Series RLC Branch  LConnTagsString=__new0  RConnTagsString=__new0  BranchType=R  Resistance=DG{4}.Y  Inductance=1e-2  SetiL0=off  InitialCurrent=0  Capacitance=2.2e-3  Setx0=off  InitialVoltage=0  Measurements=None
  Series RLC Branch13 : spsSeriesRLCBranchLib/Series RLC Branch  LConnTagsString=__new0  RConnTagsString=__new0  BranchType=L  Resistance=1  Inductance=DG{4}.L  SetiL0=off  InitialCurrent=0  Capacitance=1e-6  Setx0=off  InitialVoltage=0  Measurements=Branch current
  Series RLC Branch14 : spsSeriesRLCBranchLib/Series RLC Branch  LConnTagsString=__new0  RConnTagsString=__new0  BranchType=C  Resistance=1  Inductance=1e-2  SetiL0=off  InitialCurrent=0  Capacitance=DG{3}.C  Setx0=off  InitialVoltage=0  Measurements=None
  Series RLC Branch22 : spsSeriesRLCBranchLib/Series RLC Branch  LConnTagsString=__new0  RConnTagsString=__new0  BranchType=R  Resistance=DG{4}.R  Inductance=1e-2  SetiL0=off  InitialCurrent=0  Capacitance=2.2e-3  Setx0=off  InitialVoltage=0  Measurements=None
  Series RLC Branch24 : spsSeriesRLCBranchLib/Series RLC Branch  LConnTagsString=__new0  RConnTagsString=__new0  BranchType=R  Resistance=DG{4}.Y  Inductance=1e-2  SetiL0=off  InitialCurrent=0  Capacitance=2.2e-3  Setx0=off  InitialVoltage=0  Measurements=None
  Step : Step  Time=Current_Load_activation  SampleTime=0
  Voltage Measurement4 : spsVoltageMeasurementLib/Voltage Measurement  PhasorSimulation=off  OutputType=Complex  PSBequivalent=0
  + : PMIOPort  Side=Left
  - : PMIOPort  Port=2  Side=Right
  Vdc4 : Outport
  I4 : Outport  Port=2
  tag scope: IL4=global
  wires:
  Current Measurement8/1 -> [IL4]
  Current Measurement7/1 -> I4/1
  Voltage Measurement4/1 -> Vdc4/1
  Drive4/1 -> IGBT3/1
  Integrator2/1 -> Gain2/1
  Random Number2/1 -> Integrator2/1
  Random Number3/1 -> Integrator3/1
  Integrator3/1 -> Gain3/1
  Gain3/1 -> Product/1
  Disturbance activation/1(Out1) -> Product/2
  Product/1 -> Controlled Current Source2/1
  Gain2/1 -> Product1/1
  Disturbance activation1/1(Out1) -> Product1/2
  Product1/1 -> Controlled Voltage Source1/1
  Step/1 -> Controlled Current Source1/1
  connections:
  Controlled Current Source1/LConn1 -- Current Measurement7/LConn1 -- Breaker/RConn1 -- Series RLC Branch24/LConn1 -- Controlled Current Source2/RConn1 -- Series RLC Branch13/RConn1 -- Series RLC Branch14/LConn1
  Series RLC Branch1/RConn1 -- Controlled Current Source1/RConn1 -- -/RConn1 -- Voltage Measurement4/LConn2 -- Series RLC Branch24/RConn1 -- Controlled Voltage Source1/LConn1 -- Diode3/LConn1 -- DC Voltage Source3/LConn1
  IGBT3/LConn1 -- DC Voltage Source3/RConn1
  Current Measurement7/RConn1 -- +/RConn1 -- Voltage Measurement4/LConn1
  Diode3/RConn1 -- Series RLC Branch22/RConn1 -- IGBT3/RConn1
  Series RLC Branch1/LConn1 -- Breaker/LConn1
  Current Measurement8/RConn1 -- Controlled Current Source2/LConn1 -- Series RLC Branch13/LConn1
  Current Measurement8/LConn1 -- Series RLC Branch22/LConn1
  Controlled Voltage Source1/RConn1 -- Series RLC Branch14/RConn1

== system Simulink_DC_MG_4DGs_4Lines/Transmission Line 1 ==
  Controlled Current Source3 : spsControlledCurrentSourceLib/Controlled Current Source  Initialize=on  Source_Type=DC  Amplitude=0  Phase=0  Frequency=0  Measurements=None
  Disturbance activation : Subsystem
  Gain1 : Gain  Gain=-1/Line{1}.L
  Integrator : Integrator
  Product1 : Product
  Random Number : RandomNumber  Variance=line_variance  SampleTime=0.1
  Series RLC Branch1 : spsSeriesRLCBranchLib/Series RLC Branch  LConnTagsString=__new0  RConnTagsString=__new0  BranchType=R  Resistance=Line{2}.R  Inductance=1e-2  SetiL0=off  InitialCurrent=0  Capacitance=2.2e-3  Setx0=off  InitialVoltage=0  Measurements=None
  Series RLC Branch15 : spsSeriesRLCBranchLib/Series RLC Branch  LConnTagsString=__new0  RConnTagsString=__new0  BranchType=L  Resistance=1  Inductance=Line{1}.L  SetiL0=off  InitialCurrent=0  Capacitance=1e-6  Setx0=off  InitialVoltage=0  Measurements=Branch current
  + : PMIOPort  Side=Left
  - : PMIOPort  Port=2  Side=Right
  wires:
  Disturbance activation/1(Out1) -> Product1/2
  Product1/1 -> Controlled Current Source3/1
  Random Number/1 -> Integrator/1
  Gain1/1 -> Product1/1
  Integrator/1 -> Gain1/1
  connections:
  Series RLC Branch15/LConn1 -- +/RConn1
  Series RLC Branch1/RConn1 -- Controlled Current Source3/LConn1 -- Series RLC Branch15/RConn1
  Series RLC Branch1/LConn1 -- Controlled Current Source3/RConn1 -- -/RConn1

== system Simulink_DC_MG_4DGs_4Lines/Transmission Line 2 ==
  Controlled Current Source3 : spsControlledCurrentSourceLib/Controlled Current Source  Initialize=on  Source_Type=DC  Amplitude=0  Phase=0  Frequency=0  Measurements=None
  Disturbance activation : Subsystem
  Gain1 : Gain  Gain=-1/Line{2}.L
  Integrator : Integrator
  Product1 : Product
  Random Number : RandomNumber  Variance=line_variance  SampleTime=0.1
  Series RLC Branch1 : spsSeriesRLCBranchLib/Series RLC Branch  LConnTagsString=__new0  RConnTagsString=__new0  BranchType=R  Resistance=Line{2}.R  Inductance=1e-2  SetiL0=off  InitialCurrent=0  Capacitance=2.2e-3  Setx0=off  InitialVoltage=0  Measurements=None
  Series RLC Branch16 : spsSeriesRLCBranchLib/Series RLC Branch  LConnTagsString=__new0  RConnTagsString=__new0  BranchType=L  Resistance=1  Inductance=Line{2}.L  SetiL0=off  InitialCurrent=0  Capacitance=1e-6  Setx0=off  InitialVoltage=0  Measurements=Branch current
  + : PMIOPort  Side=Left
  - : PMIOPort  Port=2  Side=Right
  wires:
  Disturbance activation/1(Out1) -> Product1/2
  Product1/1 -> Controlled Current Source3/1
  Gain1/1 -> Product1/1
  Random Number/1 -> Integrator/1
  Integrator/1 -> Gain1/1
  connections:
  Series RLC Branch16/LConn1 -- Controlled Current Source3/RConn1 -- Series RLC Branch1/LConn1
  Series RLC Branch1/RConn1 -- Controlled Current Source3/LConn1 -- +/RConn1
  Series RLC Branch16/RConn1 -- -/RConn1

== system Simulink_DC_MG_4DGs_4Lines/Transmission Line 3 ==
  Controlled Current Source3 : spsControlledCurrentSourceLib/Controlled Current Source  Initialize=on  Source_Type=DC  Amplitude=0  Phase=0  Frequency=0  Measurements=None
  Disturbance activation : Subsystem
  Gain1 : Gain  Gain=-1/Line{3}.L
  Integrator : Integrator
  Product1 : Product
  Random Number : RandomNumber  Variance=line_variance  SampleTime=0.1
  Series RLC Branch17 : spsSeriesRLCBranchLib/Series RLC Branch  LConnTagsString=__new0  RConnTagsString=__new0  BranchType=L  Resistance=1  Inductance=Line{3}.L  SetiL0=off  InitialCurrent=0  Capacitance=1e-6  Setx0=off  InitialVoltage=0  Measurements=Branch current
  Series RLC Branch2 : spsSeriesRLCBranchLib/Series RLC Branch  LConnTagsString=__new0  RConnTagsString=__new0  BranchType=R  Resistance=Line{3}.R  Inductance=1e-2  SetiL0=off  InitialCurrent=0  Capacitance=2.2e-3  Setx0=off  InitialVoltage=0  Measurements=None
  + : PMIOPort  Side=Left
  - : PMIOPort  Port=2  Side=Right
  wires:
  Disturbance activation/1(Out1) -> Product1/2
  Product1/1 -> Controlled Current Source3/1
  Gain1/1 -> Product1/1
  Random Number/1 -> Integrator/1
  Integrator/1 -> Gain1/1
  connections:
  Series RLC Branch17/LConn1 -- Controlled Current Source3/RConn1 -- Series RLC Branch2/LConn1
  Series RLC Branch2/RConn1 -- Controlled Current Source3/LConn1 -- +/RConn1
  Series RLC Branch17/RConn1 -- -/RConn1

== system Simulink_DC_MG_4DGs_4Lines/Transmission Line4 ==
  Controlled Current Source3 : spsControlledCurrentSourceLib/Controlled Current Source  Initialize=on  Source_Type=DC  Amplitude=0  Phase=0  Frequency=0  Measurements=None
  Disturbance activation : Subsystem
  Gain1 : Gain  Gain=-1/Line{4}.L
  Integrator : Integrator
  Product1 : Product
  Random Number : RandomNumber  Variance=line_variance  SampleTime=0.1
  Series RLC Branch18 : spsSeriesRLCBranchLib/Series RLC Branch  LConnTagsString=__new0  RConnTagsString=__new0  BranchType=L  Resistance=1  Inductance=Line{4}.L  SetiL0=off  InitialCurrent=0  Capacitance=1e-6  Setx0=off  InitialVoltage=0  Measurements=Branch current
  Series RLC Branch3 : spsSeriesRLCBranchLib/Series RLC Branch  LConnTagsString=__new0  RConnTagsString=__new0  BranchType=R  Resistance=Line{4}.R  Inductance=1e-2  SetiL0=off  InitialCurrent=0  Capacitance=2.2e-3  Setx0=off  InitialVoltage=0  Measurements=None
  + : PMIOPort  Side=Left
  - : PMIOPort  Port=2  Side=Right
  wires:
  Disturbance activation/1(Out1) -> Product1/2
  Product1/1 -> Controlled Current Source3/1
  Gain1/1 -> Product1/1
  Random Number/1 -> Integrator/1
  Integrator/1 -> Gain1/1
  connections:
  Series RLC Branch18/LConn1 -- Controlled Current Source3/RConn1 -- Series RLC Branch3/LConn1
  Series RLC Branch3/RConn1 -- Controlled Current Source3/LConn1 -- +/RConn1
  Series RLC Branch18/RConn1 -- -/RConn1

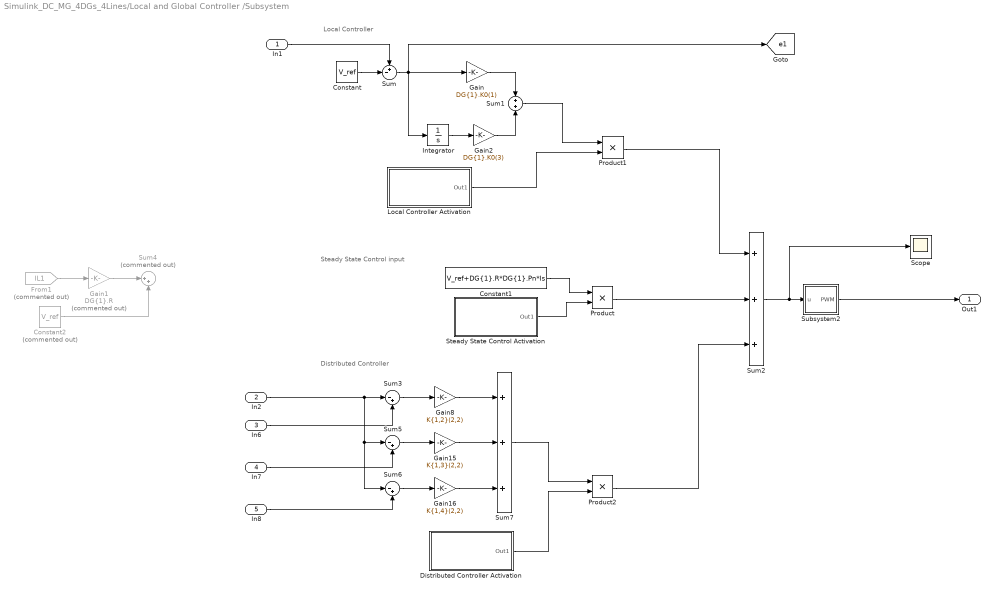
== system Simulink_DC_MG_4DGs_4Lines/Local and Global Controller /Subsystem ==
  note: Steady State Control input
  note: Local Controller
  note: Distributed Controller
  In1 : Inport
  In2 : Inport  Port=2
  In6 : Inport  Port=3
  In7 : Inport  Port=4
  In8 : Inport  Port=5
  Constant : Constant  Value=V_ref
  Constant1 : Constant  Value=V_ref+DG{1}.R*DG{1}.Pn*Is
  Constant2 : Constant  Commented=on  Value=V_ref
  Distributed Controller Activation : Subsystem
  From1 : From  Commented=on  GotoTag=IL1  TagVisibility=global
  Gain : Gain  Gain=DG{1}.K0(1)
  Gain1 : Gain  Commented=on  Gain=DG{1}.R
  Gain15 : Gain  Gain=K{1,3}(2,2)
  Gain16 : Gain  Gain=K{1,4}(2,2)
  Gain2 : Gain  Gain=DG{1}.K0(3)
  Gain8 : Gain  Gain=K{1,2}(2,2)
  Integrator : Integrator
  Local Controller Activation : Subsystem
  Product : Product
  Product1 : Product
  Product2 : Product
  Scope : Scope
  Steady State Control Activation : Subsystem
  Subsystem2 : Subsystem
      mask Display: disp('PWM')
  Sum : Sum  Inputs=+-|
  Sum1 : Sum
  Sum2 : Sum  Inputs=+++
  Sum3 : Sum  Inputs=|-+
  Sum4 : Sum  Commented=on  Inputs=|++
  Sum5 : Sum  Inputs=|-+
  Sum6 : Sum  Inputs=|-+
  Sum7 : Sum  Inputs=+++
  Out1 : Outport
  tag scope: e1=global
  wires:
  Gain/1 -> Sum1/1
  Gain2/1 -> Sum1/2
  Sum/1 -> [e1], Gain/1, Integrator/1
  In1/1 -> Sum/1
  Subsystem2/1(PWM) -> Out1/1
  Constant/1 -> Sum/2
  Integrator/1 -> Gain2/1
  Sum3/1 -> Gain8/1
  Sum5/1 -> Gain15/1
  Sum6/1 -> Gain16/1
  Gain8/1 -> Sum7/1
  Gain15/1 -> Sum7/2
  Gain16/1 -> Sum7/3
  Sum2/1 -> Scope/1, Subsystem2/1(u)
  In6/1 -> Sum3/2
  In7/1 -> Sum5/2
  In8/1 -> Sum6/2
  In2/1 -> Sum6/1, Sum5/1, Sum3/1
  Steady State Control Activation/1(Out1) -> Product/2
  Product/1 -> Sum2/2
  Sum7/1 -> Product2/1
  Distributed Controller Activation/1(Out1) -> Product2/2
  Product2/1 -> Sum2/3
  From1/1 -> Gain1/1
  Gain1/1 -> Sum4/1
  Constant2/1 -> Sum4/2
  Constant1/1 -> Product/1
  Sum1/1 -> Product1/1
  Local Controller Activation/1(Out1) -> Product1/2
  Product1/1 -> Sum2/1

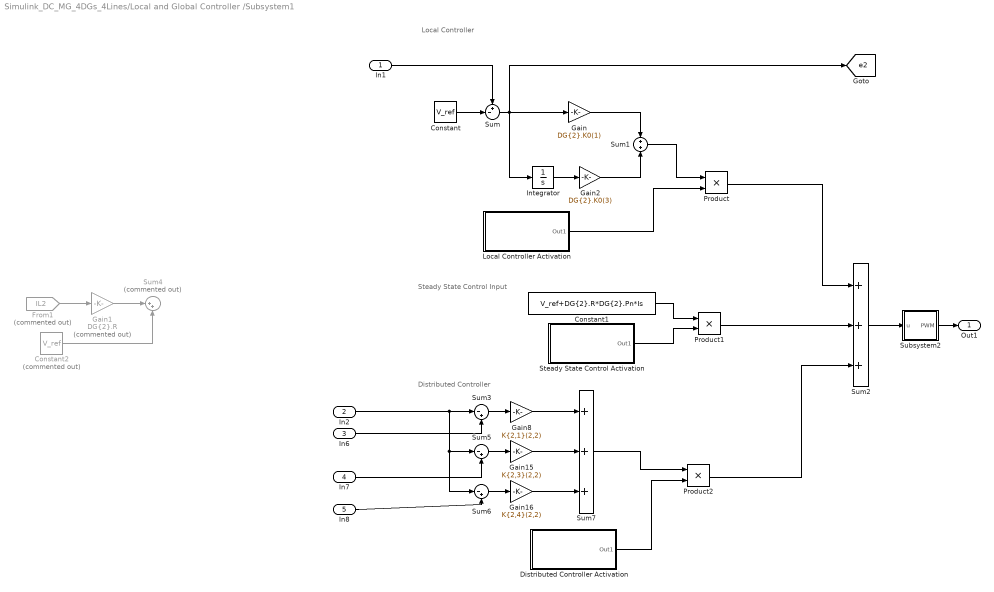
== system Simulink_DC_MG_4DGs_4Lines/Local and Global Controller /Subsystem1 ==
  note: Steady State Control Input
  note: Distributed Controller
  note: Local Controller
  In1 : Inport
  In2 : Inport  Port=2
  In6 : Inport  Port=3
  In7 : Inport  Port=4
  In8 : Inport  Port=5
  Constant : Constant  Value=V_ref
  Constant1 : Constant  Value=V_ref+DG{2}.R*DG{2}.Pn*Is
  Constant2 : Constant  Commented=on  Value=V_ref
  Distributed Controller Activation : Subsystem
  From1 : From  Commented=on  GotoTag=IL2  TagVisibility=global
  Gain : Gain  Gain=DG{2}.K0(1)
  Gain1 : Gain  Commented=on  Gain=DG{2}.R
  Gain15 : Gain  Gain=K{2,3}(2,2)
  Gain16 : Gain  Gain=K{2,4}(2,2)
  Gain2 : Gain  Gain=DG{2}.K0(3)
  Gain8 : Gain  Gain=K{2,1}(2,2)
  Integrator : Integrator
  Local Controller Activation : Subsystem
  Product : Product
  Product1 : Product
  Product2 : Product
  Steady State Control Activation : Subsystem
  Subsystem2 : Subsystem
      mask Display: disp('PWM')
  Sum : Sum  Inputs=+-|
  Sum1 : Sum
  Sum2 : Sum  Inputs=+++
  Sum3 : Sum  Inputs=|-+
  Sum4 : Sum  Commented=on  Inputs=|++
  Sum5 : Sum  Inputs=|-+
  Sum6 : Sum  Inputs=|-+
  Sum7 : Sum  Inputs=+++
  Out1 : Outport
  tag scope: e2=global
  wires:
  Gain/1 -> Sum1/1
  Gain2/1 -> Sum1/2
  Sum/1 -> Integrator/1, [e2], Gain/1
  In1/1 -> Sum/1
  Subsystem2/1(PWM) -> Out1/1
  Constant/1 -> Sum/2
  Integrator/1 -> Gain2/1
  Sum3/1 -> Gain8/1
  Sum5/1 -> Gain15/1
  Sum6/1 -> Gain16/1
  Gain8/1 -> Sum7/1
  Gain15/1 -> Sum7/2
  Gain16/1 -> Sum7/3
  Sum2/1 -> Subsystem2/1(u)
  In2/1 -> Sum6/1, Sum5/1, Sum3/1
  In6/1 -> Sum3/2
  In7/1 -> Sum5/2
  In8/1 -> Sum6/2
  Constant1/1 -> Product1/1
  Steady State Control Activation/1(Out1) -> Product1/2
  Product1/1 -> Sum2/2
  Sum7/1 -> Product2/1
  Distributed Controller Activation/1(Out1) -> Product2/2
  Product2/1 -> Sum2/3
  From1/1 -> Gain1/1
  Constant2/1 -> Sum4/2
  Gain1/1 -> Sum4/1
  Sum1/1 -> Product/1
  Local Controller Activation/1(Out1) -> Product/2
  Product/1 -> Sum2/1

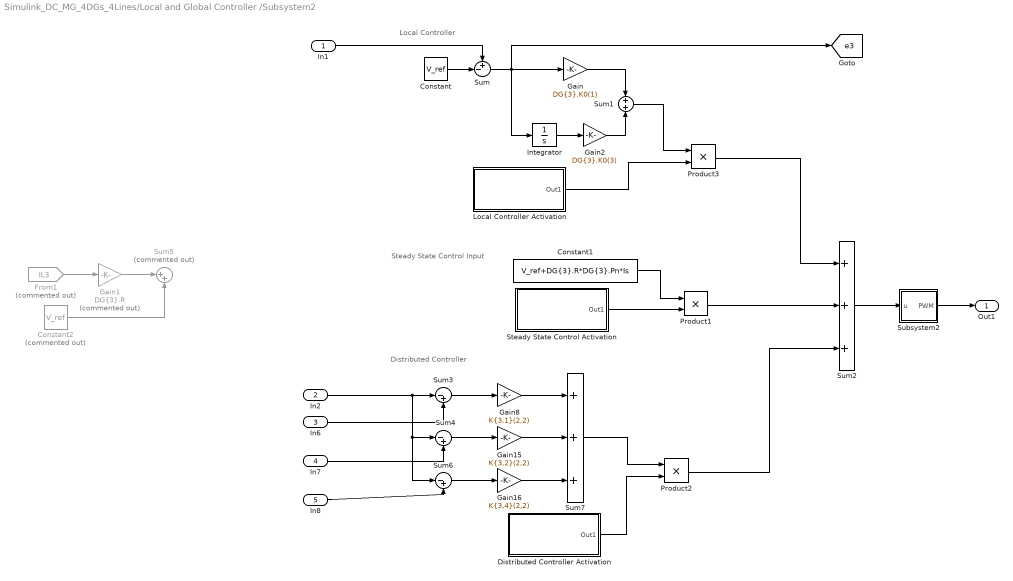
== system Simulink_DC_MG_4DGs_4Lines/Local and Global Controller /Subsystem2 ==
  note: Steady State Control Input
  note: Distributed Controller
  note: Local Controller
  In1 : Inport
  In2 : Inport  Port=2
  In6 : Inport  Port=3
  In7 : Inport  Port=4
  In8 : Inport  Port=5
  Constant : Constant  Value=V_ref
  Constant1 : Constant  Value=V_ref+DG{3}.R*DG{3}.Pn*Is
  Constant2 : Constant  Commented=on  Value=V_ref
  Distributed Controller Activation : Subsystem
  From1 : From  Commented=on  GotoTag=IL3  TagVisibility=global
  Gain : Gain  Gain=DG{3}.K0(1)
  Gain1 : Gain  Commented=on  Gain=DG{3}.R
  Gain15 : Gain  Gain=K{3,2}(2,2)
  Gain16 : Gain  Gain=K{3,4}(2,2)
  Gain2 : Gain  Gain=DG{3}.K0(3)
  Gain8 : Gain  Gain=K{3,1}(2,2)
  Integrator : Integrator
  Local Controller Activation : Subsystem
  Product1 : Product
  Product2 : Product
  Product3 : Product
  Steady State Control Activation : Subsystem
  Subsystem2 : Subsystem
      mask Display: disp('PWM')
  Sum : Sum  Inputs=+-|
  Sum1 : Sum
  Sum2 : Sum  Inputs=+++
  Sum3 : Sum  Inputs=|-+
  Sum4 : Sum  Inputs=|-+
  Sum5 : Sum  Commented=on  Inputs=|++
  Sum6 : Sum  Inputs=|-+
  Sum7 : Sum  Inputs=+++
  Out1 : Outport
  tag scope: e3=global
  wires:
  Gain2/1 -> Sum1/2
  Gain/1 -> Sum1/1
  Sum/1 -> Integrator/1, [e3], Gain/1
  In1/1 -> Sum/1
  Subsystem2/1(PWM) -> Out1/1
  Constant/1 -> Sum/2
  Integrator/1 -> Gain2/1
  Sum3/1 -> Gain8/1
  Sum4/1 -> Gain15/1
  Sum6/1 -> Gain16/1
  Gain8/1 -> Sum7/1
  Gain15/1 -> Sum7/2
  Gain16/1 -> Sum7/3
  Sum2/1 -> Subsystem2/1(u)
  In2/1 -> Sum6/1, Sum4/1, Sum3/1
  In6/1 -> Sum3/2
  In7/1 -> Sum4/2
  In8/1 -> Sum6/2
  Constant1/1 -> Product1/1
  Steady State Control Activation/1(Out1) -> Product1/2
  Product1/1 -> Sum2/2
  Sum7/1 -> Product2/1
  Distributed Controller Activation/1(Out1) -> Product2/2
  Product2/1 -> Sum2/3
  From1/1 -> Gain1/1
  Constant2/1 -> Sum5/2
  Gain1/1 -> Sum5/1
  Sum1/1 -> Product3/1
  Local Controller Activation/1(Out1) -> Product3/2
  Product3/1 -> Sum2/1

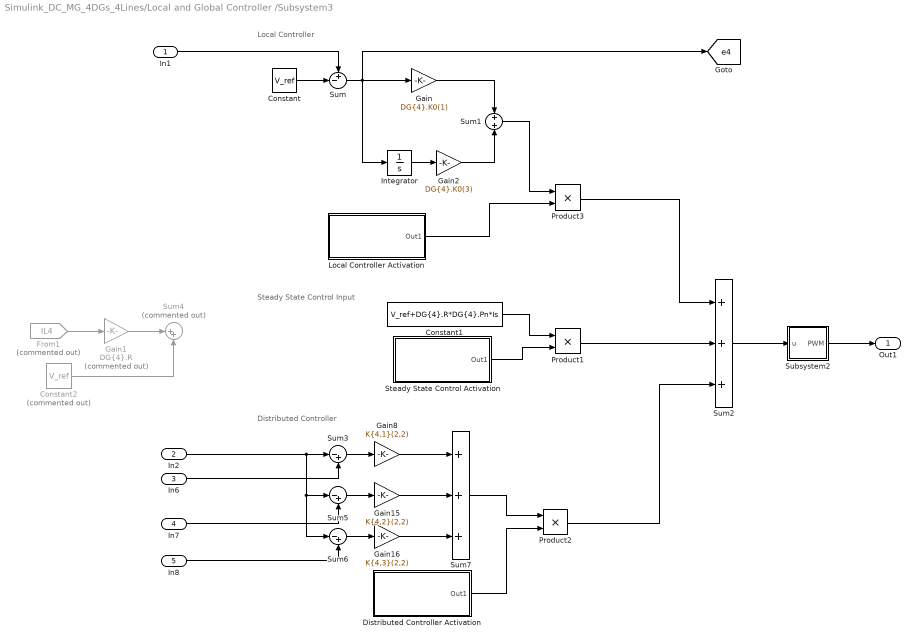
== system Simulink_DC_MG_4DGs_4Lines/Local and Global Controller /Subsystem3 ==
  note: Steady State Control Input
  note: Distributed Controller
  note: Local Controller
  In1 : Inport
  In2 : Inport  Port=2
  In6 : Inport  Port=3
  In7 : Inport  Port=4
  In8 : Inport  Port=5
  Constant : Constant  Value=V_ref
  Constant1 : Constant  Value=V_ref+DG{4}.R*DG{4}.Pn*Is
  Constant2 : Constant  Commented=on  Value=V_ref
  Distributed Controller Activation : Subsystem
  From1 : From  Commented=on  GotoTag=IL4  TagVisibility=global
  Gain : Gain  Gain=DG{4}.K0(1)
  Gain1 : Gain  Commented=on  Gain=DG{4}.R
  Gain15 : Gain  Gain=K{4,2}(2,2)
  Gain16 : Gain  Gain=K{4,3}(2,2)
  Gain2 : Gain  Gain=DG{4}.K0(3)
  Gain8 : Gain  Gain=K{4,1}(2,2)
  Integrator : Integrator
  Local Controller Activation : Subsystem
  Product1 : Product
  Product2 : Product
  Product3 : Product
  Steady State Control Activation : Subsystem
  Subsystem2 : Subsystem
      mask Display: disp('PWM')
  Sum : Sum  Inputs=+-|
  Sum1 : Sum
  Sum2 : Sum  Inputs=+++
  Sum3 : Sum  Inputs=|-+
  Sum4 : Sum  Commented=on  Inputs=|++
  Sum5 : Sum  Inputs=|-+
  Sum6 : Sum  Inputs=|-+
  Sum7 : Sum  Inputs=+++
  Out1 : Outport
  tag scope: e4=global
  wires:
  Gain/1 -> Sum1/1
  Sum/1 -> Integrator/1, [e4], Gain/1
  In1/1 -> Sum/1
  Subsystem2/1(PWM) -> Out1/1
  Constant/1 -> Sum/2
  Integrator/1 -> Gain2/1
  Sum3/1 -> Gain8/1
  Sum5/1 -> Gain15/1
  Sum6/1 -> Gain16/1
  Gain8/1 -> Sum7/1
  Gain15/1 -> Sum7/2
  Gain16/1 -> Sum7/3
  Sum2/1 -> Subsystem2/1(u)
  Gain2/1 -> Sum1/2
  In2/1 -> Sum5/1, Sum6/1, Sum3/1
  In6/1 -> Sum3/2
  In7/1 -> Sum5/2
  In8/1 -> Sum6/2
  Steady State Control Activation/1(Out1) -> Product1/2
  Constant1/1 -> Product1/1
  Product1/1 -> Sum2/2
  Distributed Controller Activation/1(Out1) -> Product2/2
  Sum7/1 -> Product2/1
  Product2/1 -> Sum2/3
  From1/1 -> Gain1/1
  Constant2/1 -> Sum4/2
  Gain1/1 -> Sum4/1
  Sum1/1 -> Product3/1
  Local Controller Activation/1(Out1) -> Product3/2
  Product3/1 -> Sum2/1

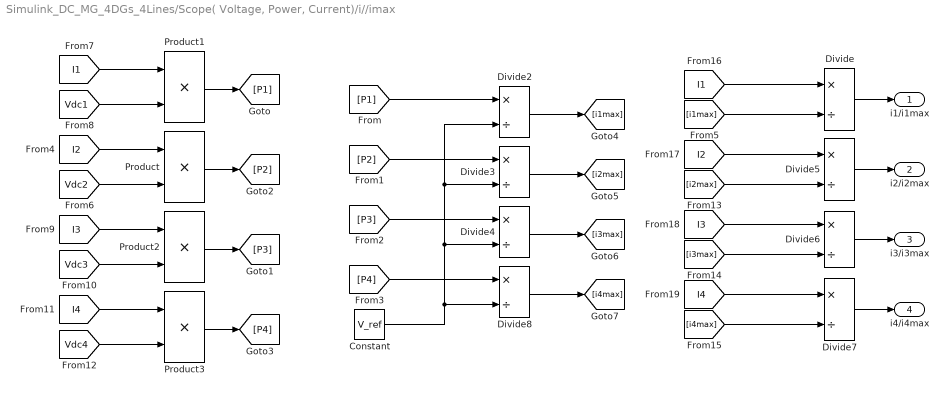
== system Simulink_DC_MG_4DGs_4Lines/Scope( Voltage, Power, Current)/i//imax ==
  Constant : Constant  Value=V_ref
  Divide{,2..8} (8 alike) : Product  Inputs=*/
  Product{,1..3} (4 alike) : Product
  i1/i1max : Outport  VectorParamsAs1DForOutWhenUnconnected=off
  i2/i2max : Outport  Port=2  VectorParamsAs1DForOutWhenUnconnected=off
  i3/i3max : Outport  Port=3  VectorParamsAs1DForOutWhenUnconnected=off
  i4/i4max : Outport  Port=4  VectorParamsAs1DForOutWhenUnconnected=off
  wires:
  Divide/1 -> i1/i1max/1
  Divide5/1 -> i2/i2max/1
  Divide6/1 -> i3/i3max/1
  Divide7/1 -> i4/i4max/1
  [Vdc3] -> Product2/2
  [Vdc1] -> Product1/2
  [Vdc2] -> Product/2
  [I1] -> Product1/1
  [I2] -> Product/1
  [Vdc4] -> Product3/2
  [I4] -> Product3/1
  [I3] -> Product2/1
  Product1/1 -> [P1]
  Product2/1 -> [P3]
  Product/1 -> [P2]
  Product3/1 -> [P4]
  [P1] -> Divide2/1
  [P2] -> Divide3/1
  [P3] -> Divide4/1
  [P4] -> Divide8/1
  Constant/1 -> Divide8/2, Divide4/2, Divide3/2, Divide2/2
  Divide8/1 -> [i4max]
  Divide4/1 -> [i3max]
  Divide3/1 -> [i2max]
  Divide2/1 -> [i1max]
  [i1max] -> Divide/2
  [i2max] -> Divide5/2
  [i3max] -> Divide6/2
  [i4max] -> Divide7/2
  [I1] -> Divide/1
  [I2] -> Divide5/1
  [I3] -> Divide6/1
  [I4] -> Divide7/1

== system Simulink_DC_MG_4DGs_4Lines/Subsystem/Breaker3 ==
  Ideal Switch : spsIdealSwitchLib/Ideal Switch  Ron=0.001  Lon=0  IC=0  Rs=1e5  Cs=inf  Measurements=on
  Stair Generator : spsStairGeneratorLib/Stair Generator  t=[0,PlugOut,PlugIn]  e=[1, 0, 1]  Ts=0
  DG3 : PMIOPort  Side=Left
  + : PMIOPort  Port=2  Side=Right
  wires:
  Stair Generator/1 -> Ideal Switch/1
  connections:
  Ideal Switch/LConn1 -- DG3/RConn1
  Ideal Switch/RConn1 -- +/RConn1

== system Simulink_DC_MG_4DGs_4Lines/Subsystem/Disturbance activation ==
  Clock : Clock
  Constant1 : Constant  Value=D_Activation
  Relational Operator : RelationalOperator  OutDataTypeStr=boolean  RndMeth=Simplest  InputSameDT=off
  Out1 : Outport  VectorParamsAs1DForOutWhenUnconnected=off
  wires:
  Clock/1 -> Relational Operator/1
  Relational Operator/1 -> Out1/1
  Constant1/1 -> Relational Operator/2

== system Simulink_DC_MG_4DGs_4Lines/Subsystem/Disturbance activation1 ==
  Clock : Clock
  Constant1 : Constant  Value=D_Activation
  Relational Operator : RelationalOperator  OutDataTypeStr=boolean  RndMeth=Simplest  InputSameDT=off
  Out1 : Outport  VectorParamsAs1DForOutWhenUnconnected=off
  wires:
  Clock/1 -> Relational Operator/1
  Relational Operator/1 -> Out1/1
  Constant1/1 -> Relational Operator/2

== system Simulink_DC_MG_4DGs_4Lines/Subsystem4/Breaker1 ==
  Ideal Switch : spsIdealSwitchLib/Ideal Switch  Ron=0.001  Lon=0  IC=0  Rs=1e5  Cs=inf  Measurements=on
  Stair Generator : spsStairGeneratorLib/Stair Generator  t=[0,PlugOut,PlugIn]  e=[1, 0, 1]  Ts=0
  DG1 : PMIOPort  Side=Left
  + : PMIOPort  Port=2  Side=Right
  wires:
  Stair Generator/1 -> Ideal Switch/1
  connections:
  Ideal Switch/RConn1 -- +/RConn1
  Ideal Switch/LConn1 -- DG1/RConn1

== system Simulink_DC_MG_4DGs_4Lines/Subsystem4/Disturbance activation ==
  Clock : Clock
  Constant1 : Constant  Value=D_Activation
  Relational Operator : RelationalOperator  OutDataTypeStr=boolean  RndMeth=Simplest  InputSameDT=off
  Out1 : Outport  VectorParamsAs1DForOutWhenUnconnected=off
  wires:
  Clock/1 -> Relational Operator/1
  Relational Operator/1 -> Out1/1
  Constant1/1 -> Relational Operator/2

== system Simulink_DC_MG_4DGs_4Lines/Subsystem4/Disturbance activation1 ==
  Clock : Clock
  Constant1 : Constant  Value=D_Activation
  Relational Operator : RelationalOperator  OutDataTypeStr=boolean  RndMeth=Simplest  InputSameDT=off
  Out1 : Outport  VectorParamsAs1DForOutWhenUnconnected=off
  wires:
  Constant1/1 -> Relational Operator/2
  Relational Operator/1 -> Out1/1
  Clock/1 -> Relational Operator/1

== system Simulink_DC_MG_4DGs_4Lines/Subsystem5/Breaker ==
  Ideal Switch : spsIdealSwitchLib/Ideal Switch  Ron=0.001  Lon=0  IC=0  Rs=1e5  Cs=inf  Measurements=on
  Stair Generator : spsStairGeneratorLib/Stair Generator  t=[0,PlugOut,PlugIn]  e=[1, 0, 1]  Ts=0
  DG2 : PMIOPort  Side=Left
  + : PMIOPort  Port=2  Side=Right
  wires:
  Stair Generator/1 -> Ideal Switch/1
  connections:
  Ideal Switch/LConn1 -- DG2/RConn1
  Ideal Switch/RConn1 -- +/RConn1

== system Simulink_DC_MG_4DGs_4Lines/Subsystem5/Disturbance activation ==
  Clock : Clock
  Constant1 : Constant  Value=D_Activation
  Relational Operator : RelationalOperator  OutDataTypeStr=boolean  RndMeth=Simplest  InputSameDT=off
  Out1 : Outport  VectorParamsAs1DForOutWhenUnconnected=off
  wires:
  Clock/1 -> Relational Operator/1
  Relational Operator/1 -> Out1/1
  Constant1/1 -> Relational Operator/2

== system Simulink_DC_MG_4DGs_4Lines/Subsystem5/Disturbance activation1 ==
  Clock : Clock
  Constant1 : Constant  Value=D_Activation
  Relational Operator : RelationalOperator  OutDataTypeStr=boolean  RndMeth=Simplest  InputSameDT=off
  Out1 : Outport  VectorParamsAs1DForOutWhenUnconnected=off
  wires:
  Constant1/1 -> Relational Operator/2
  Relational Operator/1 -> Out1/1
  Clock/1 -> Relational Operator/1

== system Simulink_DC_MG_4DGs_4Lines/Subsystem6/Breaker ==
  Ideal Switch : spsIdealSwitchLib/Ideal Switch  Ron=0.001  Lon=0  IC=0  Rs=1e5  Cs=inf  Measurements=on
  Stair Generator : spsStairGeneratorLib/Stair Generator  t=[0,PlugOut,PlugIn]  e=[1, 0, 1]  Ts=0
  DG4 : PMIOPort  Side=Left
  + : PMIOPort  Port=2  Side=Right
  wires:
  Stair Generator/1 -> Ideal Switch/1
  connections:
  Ideal Switch/LConn1 -- DG4/RConn1
  Ideal Switch/RConn1 -- +/RConn1

== system Simulink_DC_MG_4DGs_4Lines/Subsystem6/Disturbance activation ==
  Clock : Clock
  Constant1 : Constant  Value=D_Activation
  Relational Operator : RelationalOperator  OutDataTypeStr=boolean  RndMeth=Simplest  InputSameDT=off
  Out1 : Outport  VectorParamsAs1DForOutWhenUnconnected=off
  wires:
  Clock/1 -> Relational Operator/1
  Relational Operator/1 -> Out1/1
  Constant1/1 -> Relational Operator/2
